simulink model "Individual_1"  (R2026b)
settings: Solver=VariableStepAuto
settings Model: Creator=David  LastModifiedBy=David

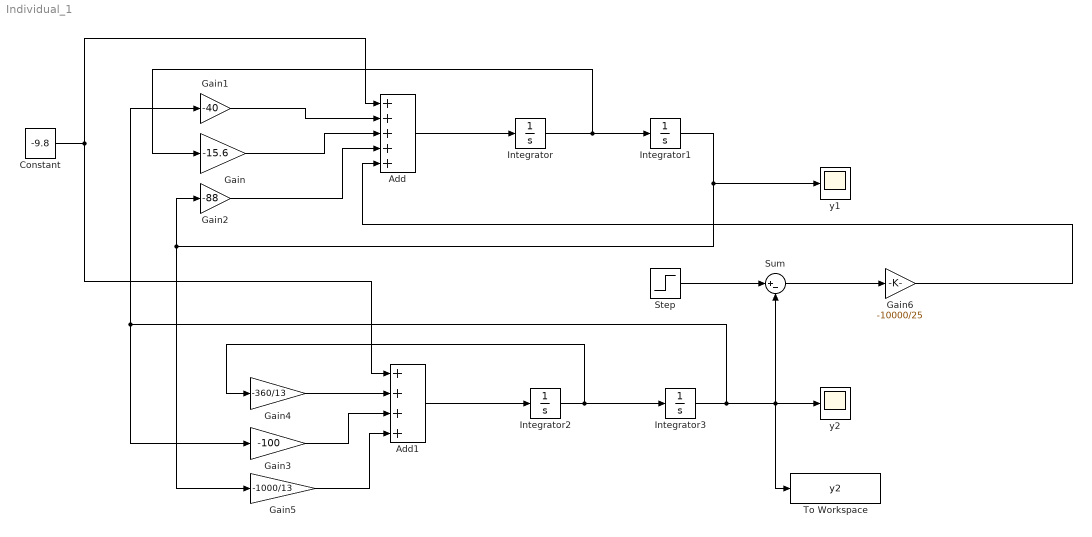
== system Individual_1 ==
  Add : Sum  Inputs=+++++
  Add1 : Sum  Inputs=++++
  Constant : Constant  Value=-9.8
  Gain : Gain  Gain=-15.6
  Gain1 : Gain  Gain=-40
  Gain2 : Gain  Gain=-88
  Gain3 : Gain  Gain=-100
  Gain4 : Gain  Gain=-360/13
  Gain5 : Gain  Gain=-1000/13
  Gain6 : Gain  Gain=-10000/25
  Integrator{,1..3} (4 alike) : Integrator
  Step : Step  Time=0  FinalValue=5  SampleTime=0
  Sum : Sum  Inputs=|+-
  To Workspace : ToWorkspace  VariableName=y2  SaveFormat=Timeseries  SampleTime=-1
  y1 : Scope
      settings: ActiveDisplayYMinimum=-1.2758873826570503E+11  ActiveDisplayYMaximum=-6.285724392531356E+10
  y2 : Scope
      settings: ActiveDisplayYMinimum=4.2728760743266667  ActiveDisplayYMaximum=4.3748942074367481
  wires:
  Add/1 -> Integrator/1
  Gain2/1 -> Add/4
  Constant/1 -> Add/1, Add1/1
  Integrator2/1 -> Gain4/1, Integrator3/1
  Gain6/1 -> Add/5
  Gain4/1 -> Add1/2
  Add1/1 -> Integrator2/1
  Gain5/1 -> Add1/4
  Integrator1/1 -> Gain2/1, Gain5/1, y1/1
  Integrator3/1 -> Gain3/1, Gain1/1, To Workspace/1, y2/1, Sum/2
  Gain/1 -> Add/3
  Gain3/1 -> Add1/3
  Sum/1 -> Gain6/1
  Step/1 -> Sum/1
  Gain1/1 -> Add/2
  Integrator/1 -> Integrator1/1, Gain/1
